simulink model "Model_31_03_2"  (R2024b)
settings: Solver=ode4  StartTime=0.0  StopTime=100  FixedStep=0.1  RelTol=1e-3
values from neighbouring files (symbols this model uses):
  A = [Xu Xw-q_trim -w_trim -g*cos(theta_trim*pi/180) 0 ... (first row only)    [Code_31_03.m]
  B = [Xde Xt; Zde Zt; Mde Mt; 0 0; 0 0]    [Code_31_03.m]
  diff_delta_e = -1    [Code_31_03.m]
  x0 = [0;0;0;0;0]    [Code_31_03.m]
  x0_ver_lin = [61.7334;0.9051;0;0.84*pi/180; 0]    [Code_31_03.m]
settings Model: Creator=baron  LastModifiedBy=baron

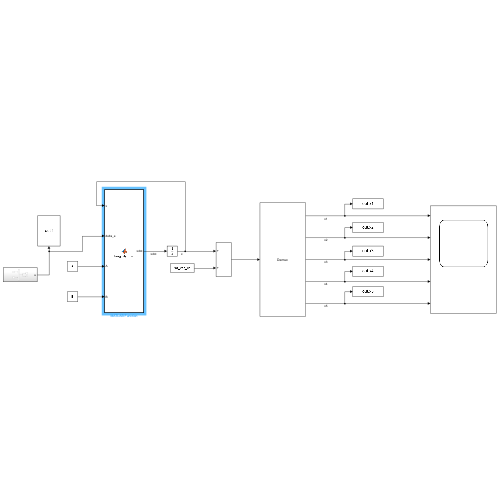
[thumbnail: Simulink's stored preview of the top-level diagram]
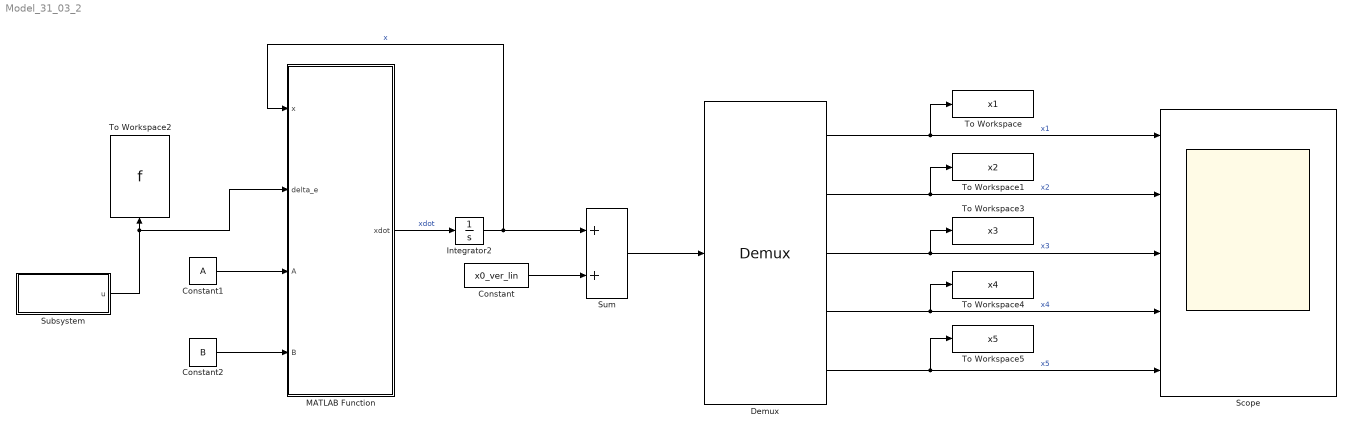
== system Model_31_03_2 ==
  Constant : Constant  Value=x0_ver_lin
  Constant1 : Constant  Value=A
  Constant2 : Constant  Value=B
  Demux : Demux  Outputs=5
      settings: DisplayOption=none
  Integrator2 : Integrator  InitialCondition=x0
  MATLAB Function : MATLAB Function  TreatAsAtomicUnit=on
  Scope : Scope  NumInputPorts=5
  Subsystem : Subsystem
  Sum : Sum
  To Workspace : ToWorkspace  VariableName=x1  SampleTime=-1
      settings: Save2DSignal=2-D array (concatenate along first dimension)
  To Workspace1 : ToWorkspace  VariableName=x2  SampleTime=-1
      settings: Save2DSignal=2-D array (concatenate along first dimension)
  To Workspace2 : ToWorkspace  VariableName=f  SampleTime=-1
      settings: Save2DSignal=2-D array (concatenate along first dimension)
  To Workspace3 : ToWorkspace  VariableName=x3  SampleTime=-1
      settings: Save2DSignal=2-D array (concatenate along first dimension)
  To Workspace4 : ToWorkspace  VariableName=x4  SampleTime=-1
      settings: Save2DSignal=2-D array (concatenate along first dimension)
  To Workspace5 : ToWorkspace  VariableName=x5  SampleTime=-1
      settings: Save2DSignal=2-D array (concatenate along first dimension)
  wires:
  Integrator2/1 -> MATLAB Function/1(x), Sum/1  "x"
  MATLAB Function/1(xdot) -> Integrator2/1  "xdot"
  Demux/1 -> To Workspace/1, Scope/1  "x1"
  Demux/3 -> Scope/3, To Workspace3/1  "x3"
  Demux/4 -> Scope/4, To Workspace4/1  "x4"
  Demux/2 -> Scope/2, To Workspace1/1  "x2"
  Demux/5 -> Scope/5, To Workspace5/1  "x5"
  Subsystem/1(u) -> MATLAB Function/2(delta_e), To Workspace2/1
  Sum/1 -> Demux/1
  Constant/1 -> Sum/2
  Constant1/1 -> MATLAB Function/3(A)
  Constant2/1 -> MATLAB Function/4(B)

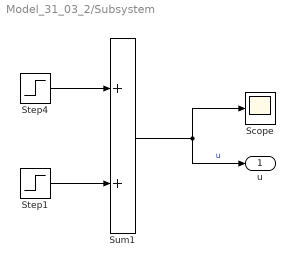
== system Model_31_03_2/Subsystem ==
  Scope : Scope
  Step1 : Step  Time=10  After=-diff_delta_e*pi/180  SampleTime=0
  Step4 : Step  Time=5  After=(diff_delta_e)*pi/180  SampleTime=0
  Sum1 : Sum
  u : Outport
  wires:
  Sum1/1 -> u/1, Scope/1  "u"
  Step4/1 -> Sum1/1
  Step1/1 -> Sum1/2

== matlab function Model_31_03_2/MATLAB Function ==
  data: x input; xdot output; delta_e input; A input; B input
function xdot  = long_dyn_lin(x,delta_e,A,B)
    
    xdot = A*x + B*[delta_e; 0];

end
